simulink model "Exp5"  (R2025b)
settings: Solver=VariableStepAuto  StartTime=0.0  StopTime=10.0  RelTol=1e-3
libraries: simulink x4
settings Model: Creator=SUBHASH  LastModifiedBy=SUBHASH

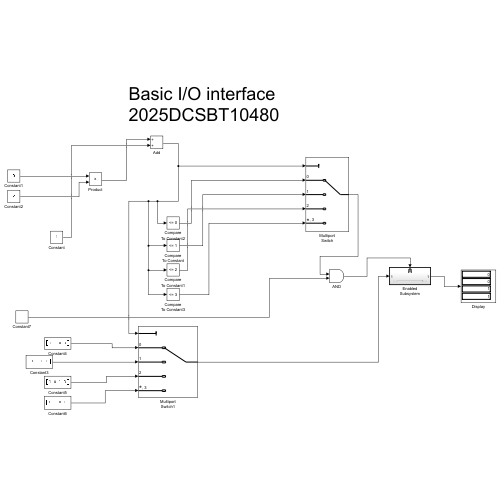
[thumbnail: Simulink's stored preview of the top-level diagram]
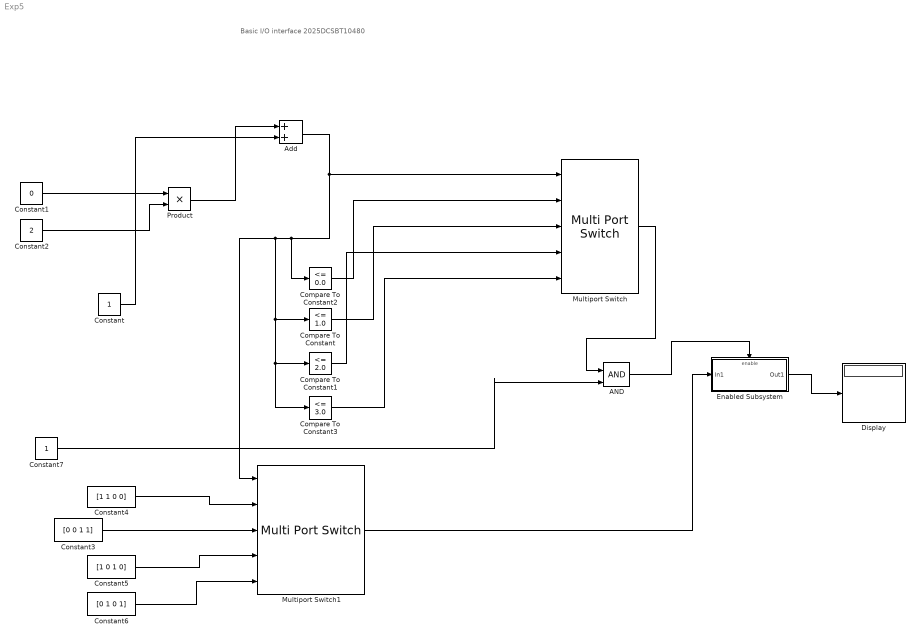
== system Exp5 ==
  note: Basic I/O interface
      | 2025DCSBT10480
  AND : Logic  IconShape=distinctive  AllPortsSameDT=off  OutDataTypeStr=boolean
  Add : Sum
  Compare To Constant : simulink/Logic and Bit Operations/Compare To Constant  relop=<=  const=1.0  OutDataTypeStr=boolean
  Compare To Constant1 : simulink/Logic and Bit Operations/Compare To Constant  relop=<=  const=2.0  OutDataTypeStr=boolean
  Compare To Constant2 : simulink/Logic and Bit Operations/Compare To Constant  relop=<=  const=0.0  OutDataTypeStr=boolean
  Compare To Constant3 : simulink/Logic and Bit Operations/Compare To Constant  relop=<=  const=3.0  OutDataTypeStr=boolean
  Constant : Constant
  Constant1 : Constant  Value=0
  Constant2 : Constant  Value=2
  Constant3 : Constant  Value=[0 0 1 1]
  Constant4 : Constant  Value=[1 1 0 0]
  Constant5 : Constant  Value=[1 0 1 0]
  Constant6 : Constant  Value=[0 1 0 1]
  Constant7 : Constant
  Display : Display
  Enabled Subsystem : Subsystem  TreatAsAtomicUnit=on
  Multiport Switch : MultiPortSwitch  DataPortOrder=Zero-based contiguous  Inputs=4  zeroidx=on  SaturateOnIntegerOverflow=off  InputSameDT=off
  Multiport Switch1 : MultiPortSwitch  DataPortOrder=Zero-based contiguous  Inputs=4  zeroidx=on  SaturateOnIntegerOverflow=off  InputSameDT=off
  Product : Product
  wires:
  Constant1/1 -> Product/1
  Constant2/1 -> Product/2
  Constant/1 -> Add/2
  Product/1 -> Add/1
  AND/1 -> Enabled Subsystem/Enable
  Multiport Switch1/1 -> Enabled Subsystem/1(In1)
  Constant4/1 -> Multiport Switch1/2
  Constant3/1 -> Multiport Switch1/3
  Constant5/1 -> Multiport Switch1/4
  Constant6/1 -> Multiport Switch1/5
  Constant7/1 -> AND/2
  Add/1 -> Multiport Switch1/1, Compare To Constant3/1, Compare To Constant1/1, Compare To Constant/1, Compare To Constant2/1, Multiport Switch/1
  Compare To Constant/1 -> Multiport Switch/3
  Compare To Constant2/1 -> Multiport Switch/2
  Compare To Constant1/1 -> Multiport Switch/4
  Compare To Constant3/1 -> Multiport Switch/5
  Enabled Subsystem/1(Out1) -> Display/1
  Multiport Switch/1 -> AND/1

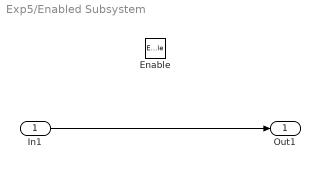
== system Exp5/Enabled Subsystem ==
  In1 : Inport
  Enable : EnablePort
  Out1 : Outport
  wires:
  In1/1 -> Out1/1
